simulink model "voltage_sensor"  (R2026a)
settings: Solver=VariableStepAuto
libraries: fl_lib x2, nesl_utility x1
settings Model: Creator=Fer Alexandru  LastModifiedBy=Fer Alexandru

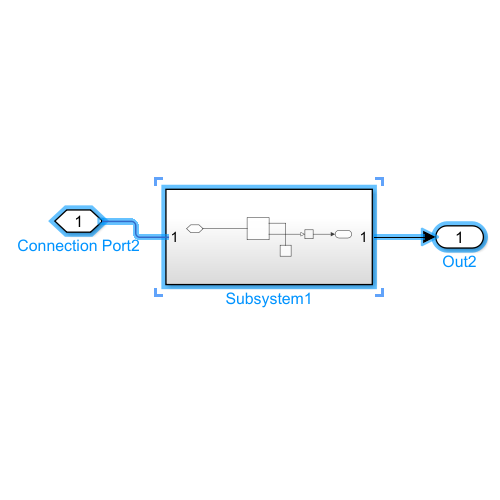
[thumbnail: Simulink's stored preview of the top-level diagram]
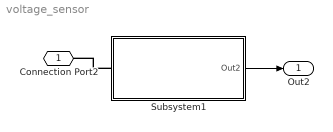
== system voltage_sensor ==
  Subsystem1 : Subsystem
  Connection Port2 : PMIOPort  Side=Left
  Out2 : Outport
  wires:
  Subsystem1/1(Out2) -> Out2/1
  connections:
  Subsystem1/LConn1 -- Connection Port2/RConn1

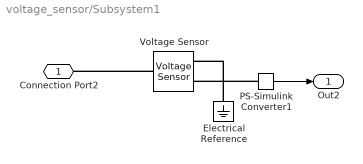
== system voltage_sensor/Subsystem1 ==
  Electrical Reference : fl_lib/Electrical/Electrical Elements/Electrical Reference
  PS-Simulink Converter1 : nesl_utility/PS-Simulink Converter  PhysicalDomain=network_engine_domain  SubClassName=ps_output  LeftPortType=input  RightPortType=output  PseudoPeriodic=off  Frequencies=[]  VectorFormat=inherit  Unit=inherit  AffineConversion=off
  Voltage Sensor : fl_lib/Electrical/Electrical Sensors/Voltage Sensor
  Connection Port2 : PMIOPort  Side=Left
  Out2 : Outport
  wires:
  PS-Simulink Converter1/1 -> Out2/1
  connections:
  Voltage Sensor/LConn1 -- Connection Port2/RConn1
  PS-Simulink Converter1/LConn1 -- Voltage Sensor/RConn1
  Electrical Reference/LConn1 -- Voltage Sensor/RConn2
